simulink library "three_phase_rlc_load"  (R2025b)
settings: Solver=VariableStepAuto  StartTime=0.0  StopTime=10.0  RelTol=1e-3
libraries: fl_lib x6
settings Model: Creator=ltnbda  LastModifiedBy=dbagn

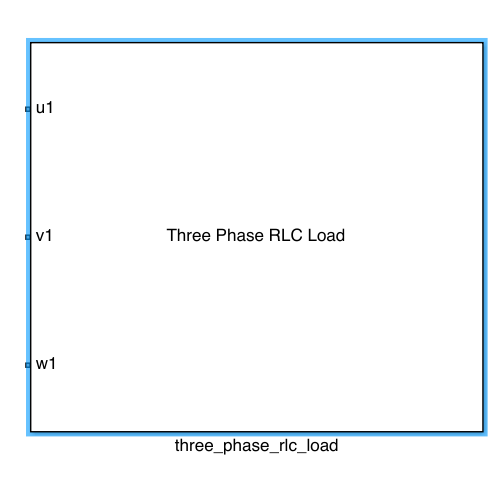
[thumbnail: Simulink's stored preview of the top-level diagram]
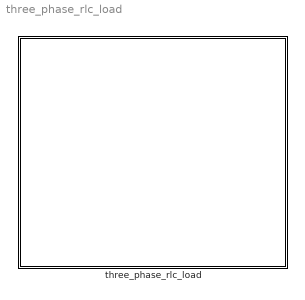
== system three_phase_rlc_load ==
  three_phase_rlc_load : Subsystem  mask{Ls_load=1e-3, Cs_load=1e-3, Rs_load=1}
      mask prompts: Ls_load "Ls_load (H)"; Cs_load "Cs_load (F)"; Rs_load "Rs_load (Ohm)"
      mask Display:
      | disp('Three Phase RLC Load');
      | port_label('lconn', 1, 'u1');
      | port_label('lconn', 2, 'v1');
      | port_label('lconn', 3, 'w1');

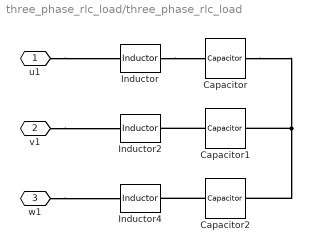
== system three_phase_rlc_load/three_phase_rlc_load ==
  Capacitor : fl_lib/Electrical/Electrical Elements/Capacitor  c=Cs_load F  r=1e-6 Ohm  g=0 1/Ohm  i_specify=off  i_priority=None  i=0 A  i_nominal_specify=off  i_nominal_value=1  i_nominal_unit=A  v_specify=off  v_priority=None  v=0 V  v_nominal_specify=off  v_nominal_value=1  v_nominal_unit=V  vc_specify=off  vc_priority=High  vc=0 V  vc_nominal_specify=off  vc_nominal_value=1  vc_nominal_unit=V
  Capacitor1 : fl_lib/Electrical/Electrical Elements/Capacitor  c=Cs_load F  r=1e-6 Ohm  g=0 1/Ohm  i_specify=off  i_priority=None  i=0 A  i_nominal_specify=off  i_nominal_value=1  i_nominal_unit=A  v_specify=off  v_priority=None  v=0 V  v_nominal_specify=off  v_nominal_value=1  v_nominal_unit=V  vc_specify=off  vc_priority=High  vc=0 V  vc_nominal_specify=off  vc_nominal_value=1  vc_nominal_unit=V
  Capacitor2 : fl_lib/Electrical/Electrical Elements/Capacitor  c=Cs_load F  r=1e-6 Ohm  g=0 1/Ohm  i_specify=off  i_priority=None  i=0 A  i_nominal_specify=off  i_nominal_value=1  i_nominal_unit=A  v_specify=off  v_priority=None  v=0 V  v_nominal_specify=off  v_nominal_value=1  v_nominal_unit=V  vc_specify=off  vc_priority=High  vc=0 V  vc_nominal_specify=off  vc_nominal_value=1  vc_nominal_unit=V
  Inductor : fl_lib/Electrical/Electrical Elements/Inductor  l=Ls_load H  r=Rs_load Ohm  g=1e-9 1/Ohm  i_specify=off  i_priority=None  i=0 A  i_nominal_specify=off  i_nominal_value=1  i_nominal_unit=A  v_specify=off  v_priority=None  v=0 V  v_nominal_specify=off  v_nominal_value=1  v_nominal_unit=V  i_L_specify=off  i_L_priority=High  i_L=0 A  i_L_nominal_specify=off  i_L_nominal_value=1  i_L_nominal_unit=A
  Inductor2 : fl_lib/Electrical/Electrical Elements/Inductor  l=Ls_load H  r=Rs_load Ohm  g=1e-9 1/Ohm  i_specify=off  i_priority=None  i=0 A  i_nominal_specify=off  i_nominal_value=1  i_nominal_unit=A  v_specify=off  v_priority=None  v=0 V  v_nominal_specify=off  v_nominal_value=1  v_nominal_unit=V  i_L_specify=off  i_L_priority=High  i_L=0 A  i_L_nominal_specify=off  i_L_nominal_value=1  i_L_nominal_unit=A
  Inductor4 : fl_lib/Electrical/Electrical Elements/Inductor  l=Ls_load H  r=Rs_load Ohm  g=1e-9 1/Ohm  i_specify=off  i_priority=None  i=0 A  i_nominal_specify=off  i_nominal_value=1  i_nominal_unit=A  v_specify=off  v_priority=None  v=0 V  v_nominal_specify=off  v_nominal_value=1  v_nominal_unit=V  i_L_specify=off  i_L_priority=High  i_L=0 A  i_L_nominal_specify=off  i_L_nominal_value=1  i_L_nominal_unit=A
  u1 : PMIOPort  Side=Left
  v1 : PMIOPort  Port=2  Side=Left
  w1 : PMIOPort  Port=3  Side=Left
  connections:
  u1/RConn1 -- Inductor/LConn1
  w1/RConn1 -- Inductor4/LConn1
  v1/RConn1 -- Inductor2/LConn1
  Inductor/RConn1 -- Capacitor/LConn1
  Capacitor1/LConn1 -- Inductor2/RConn1
  Capacitor/RConn1 -- Capacitor1/RConn1 -- Capacitor2/RConn1
  Capacitor2/LConn1 -- Inductor4/RConn1
